simulink model "emso2"  (Simulink 7.1)
settings: Solver=VariableStepDiscrete  StartTime=0.0  StopTime=2  RelTol=1e-3
settings Model: Creator=lades  LastModifiedBy=Administrator
settings DataIOCC: ExternalInput=Az

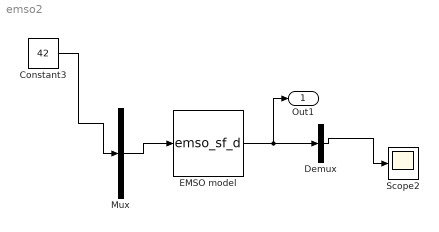
== system emso2 ==
  Constant3 : Constant  Value=42  OutDataType=sfix(16)  OutScaling=2^0
  Demux : Demux  Outputs=1
  EMSO model : S-Function  FunctionName=emso_sf_d  Parameters='pg.ems',1,1,0.5  EnableBusSupport=off
  Mux : Mux  Inputs=1
  Scope2 : Scope
      settings: TimeRange=2  YMin=26  YMax=28  SaveName=ScopeData2
  Out1 : Outport  OutDataType=sfix(16)  OutScaling=2^0
  wires:
  EMSO model/1 -> Out1/1, Demux/1
  Constant3/1 -> Mux/1
  Mux/1 -> EMSO model/1
  Demux/1 -> Scope2/1
